simulink model "VSG_AdaptiveJD"  (R2023b)
settings: Solver=ode4  StartTime=0  StopTime=Tsim  FixedStep=Ts  RelTol=1e-3
InitFcn:
  | p0 = fileparts(get_param(bdroot, 'FileName'));
  | if ~isempty(p0), addpath(p0);
  | end;
  | if ~exist('VSG_CASE', 'var'),
  |     VSG_CASE = 'case1';
  | end;
  | if ~exist('VSG_SCHEME', 'var'),
  |     VSG_SCHEME = 5;
  | end;
  | init_vsg_params(VSG_CASE, VSG_SCHEME);
undefined symbols (not defined in the file or in its folder): a_n, b_n, db, delta0, dfref, Dmax, Dmin, dref, DS0, dwref, dzd, dzr, J0, Jmax, Jmin, Kd, kpsi, Kw, lam, lam_floor, muJ, nb, nu, qref, scheme, sigma_n, tau, Ts, txi, w0, wn0, z0, zmax
Description:
  | VSG 转动惯量与阻尼系数协同自适应控制（闭环指标整形, MSCA）
  | 定步长 ode4, Ts = 2e-4 s，与 git/vsg_sim5.py 数值一致。
  | 参数见 init_vsg_params.m；run_vsg_slx.m 复现三工况五方案结果。
settings Model: Creator=Lenovo  LastModifiedBy=Lenovo

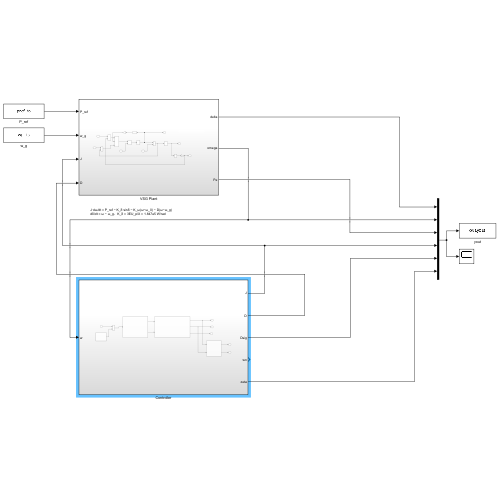
[thumbnail: Simulink's stored preview of the top-level diagram]
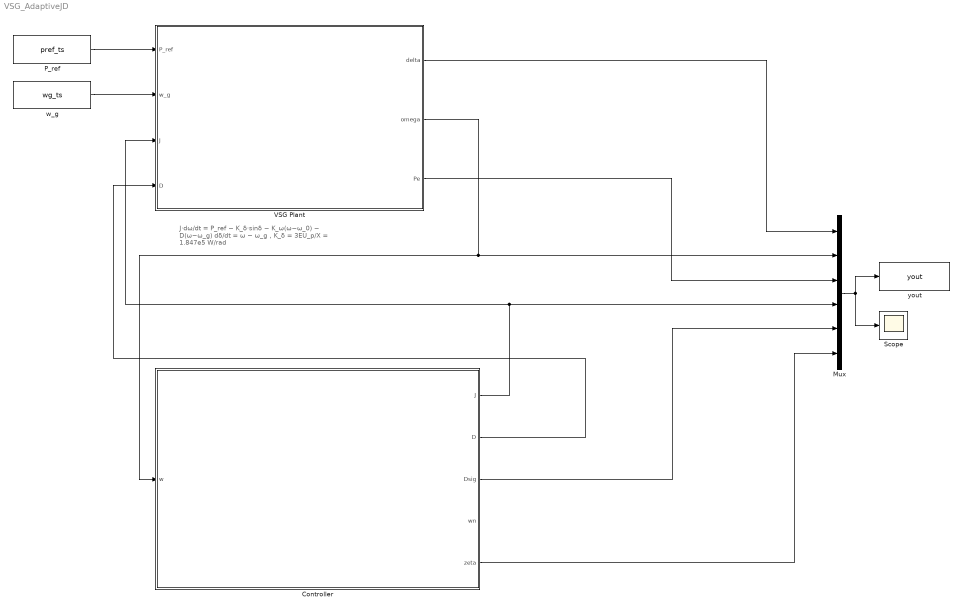
== system VSG_AdaptiveJD ==
  note: J·dω/dt = P_ref − K_δ·sinδ − K_ω(ω−ω_0) − D(ω−ω_g)
      | dδ/dt = ω − ω_g，K_δ = 3EU_p/X = 1.847e5 W/rad
  Controller : Subsystem
  Mux : Mux  Inputs=6
  P_ref : FromWorkspace  VariableName=pref_ts  Interpolate=off  OutputAfterFinalValue=Holding final value
  Scope : Scope
  VSG Plant : Subsystem
  w_g : FromWorkspace  VariableName=wg_ts  Interpolate=off  OutputAfterFinalValue=Holding final value
  yout : ToWorkspace  VariableName=yout  SaveFormat=Timeseries  SampleTime=Ts
  wires:
  P_ref/1 -> VSG Plant/1(P_ref)
  w_g/1 -> VSG Plant/2(w_g)
  VSG Plant/2(omega) -> Controller/1(w), Mux/2
  Controller/1(J) -> VSG Plant/3(J), Mux/4
  Controller/2(D) -> VSG Plant/4(D)
  VSG Plant/1(delta) -> Mux/1
  VSG Plant/3(Pe) -> Mux/3
  Controller/3(Dsig) -> Mux/5
  Controller/5(zeta) -> Mux/6
  Mux/1 -> yout/1, Scope/1

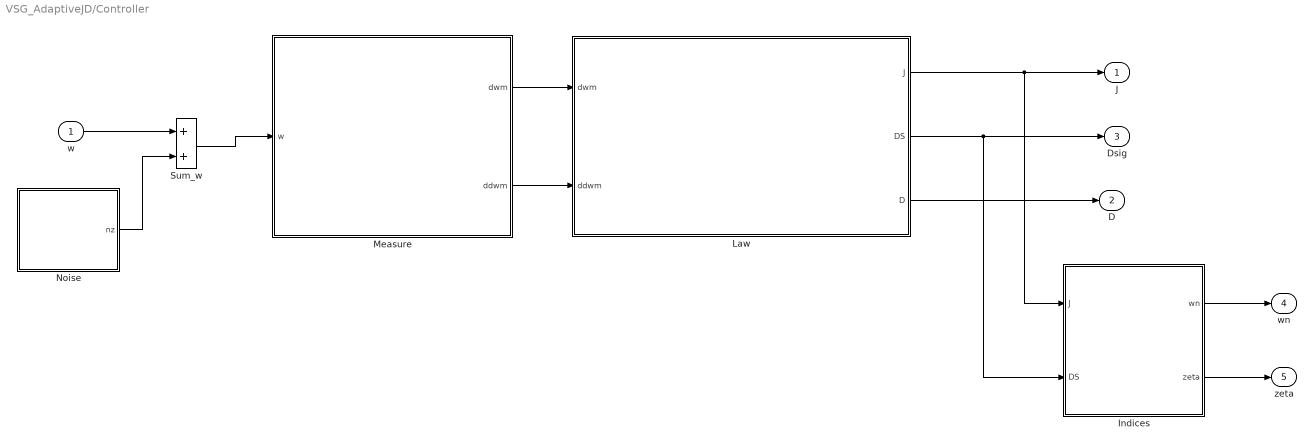
== system VSG_AdaptiveJD/Controller ==
  w : Inport
  Indices : Subsystem
  Law : Subsystem
  Measure : Subsystem
  Noise : Subsystem
  Sum_w : Sum
  J : Outport
  D : Outport  Port=2
  Dsig : Outport  Port=3
  wn : Outport  Port=4
  zeta : Outport  Port=5
  wires:
  w/1 -> Sum_w/1
  Noise/1(nz) -> Sum_w/2
  Sum_w/1 -> Measure/1(w)
  Measure/1(dwm) -> Law/1(dwm)
  Measure/2(ddwm) -> Law/2(ddwm)
  Law/1(J) -> J/1, Indices/1(J)
  Law/2(DS) -> Indices/2(DS), Dsig/1
  Law/3(D) -> D/1
  Indices/1(wn) -> wn/1
  Indices/2(zeta) -> zeta/1

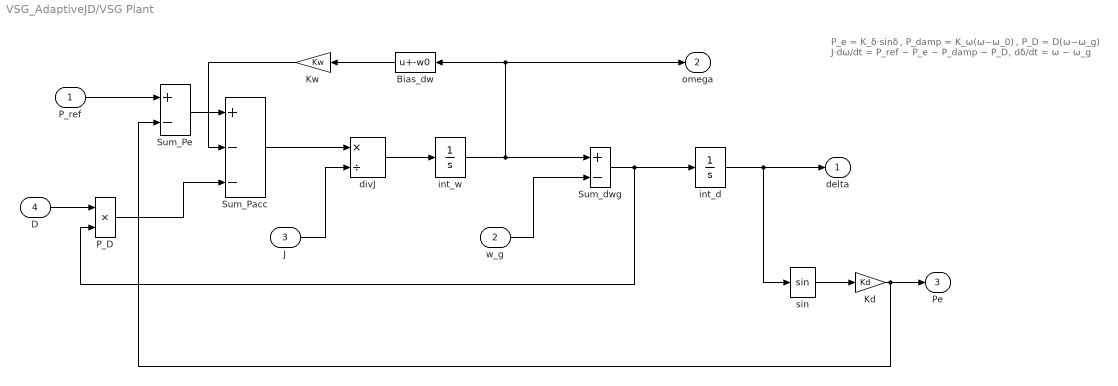
== system VSG_AdaptiveJD/VSG Plant ==
  note: P_e = K_δ·sinδ，P_damp = K_ω(ω−ω_0)，P_D = D(ω−ω_g)
      | J·dω/dt = P_ref − P_e − P_damp − P_D，dδ/dt = ω − ω_g
  P_ref : Inport
  w_g : Inport  Port=2
  J : Inport  Port=3
  D : Inport  Port=4
  Bias_dw : Bias  Bias=-w0  SaturateOnIntegerOverflow=off
  Kd : Gain  Gain=Kd
  Kw : Gain  Gain=Kw
  P_D : Product
  Sum_Pacc : Sum  Inputs=+--
  Sum_Pe : Sum  Inputs=+-
  Sum_dwg : Sum  Inputs=+-
  divJ : Product  Inputs=*/
  int_d : Integrator  InitialCondition=delta0
  int_w : Integrator  InitialCondition=w0
  sin : Trigonometry
  delta : Outport
  omega : Outport  Port=2
  Pe : Outport  Port=3
  wires:
  P_ref/1 -> Sum_Pe/1
  Kd/1 -> Sum_Pe/2, Pe/1
  Sum_Pe/1 -> Sum_Pacc/1
  Kw/1 -> Sum_Pacc/2
  P_D/1 -> Sum_Pacc/3
  Sum_Pacc/1 -> divJ/1
  J/1 -> divJ/2
  divJ/1 -> int_w/1
  int_w/1 -> omega/1, Bias_dw/1, Sum_dwg/1
  Bias_dw/1 -> Kw/1
  w_g/1 -> Sum_dwg/2
  Sum_dwg/1 -> int_d/1, P_D/2
  int_d/1 -> sin/1, delta/1
  sin/1 -> Kd/1
  D/1 -> P_D/1

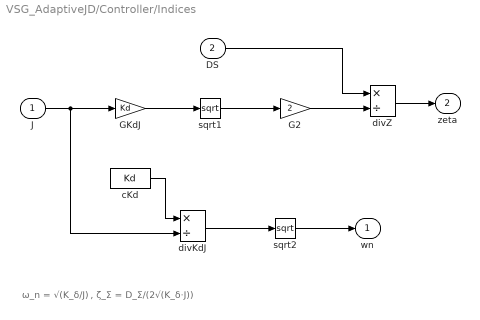
== system VSG_AdaptiveJD/Controller/Indices ==
  note: ω_n = √(K_δ/J)，ζ_Σ = D_Σ/(2√(K_δ·J))
  J : Inport
  DS : Inport  Port=2
  G2 : Gain  Gain=2
  GKdJ : Gain  Gain=Kd
  cKd : Constant  Value=Kd
  divKdJ : Product  Inputs=*/
  divZ : Product  Inputs=*/
  sqrt1 : Sqrt
  sqrt2 : Sqrt
  wn : Outport
  zeta : Outport  Port=2
  wires:
  J/1 -> GKdJ/1, divKdJ/2
  GKdJ/1 -> sqrt1/1
  sqrt1/1 -> G2/1
  cKd/1 -> divKdJ/1
  divKdJ/1 -> sqrt2/1
  sqrt2/1 -> wn/1
  DS/1 -> divZ/1
  G2/1 -> divZ/2
  divZ/1 -> zeta/1

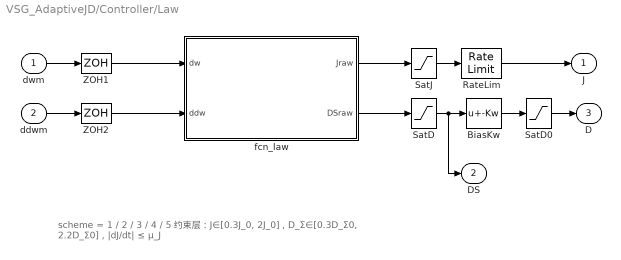
== system VSG_AdaptiveJD/Controller/Law ==
  note: scheme = 1  / 2  / 3  / 4  / 5
      | 约束层：J∈[0.3J_0, 2J_0]，D_Σ∈[0.3D_Σ0, 2.2D_Σ0]，|dJ/dt| ≤ μ_J
  dwm : Inport
  ddwm : Inport  Port=2
  BiasKw : Bias  Bias=-Kw  SaturateOnIntegerOverflow=off
  RateLim : RateLimiter  RisingSlewLimit=muJ  FallingSlewLimit=-muJ  SampleTimeMode=inherited  InitialCondition=J0
  SatD : Saturate  UpperLimit=Dmax  LowerLimit=Dmin
  SatD0 : Saturate  UpperLimit=inf  LowerLimit=0
  SatJ : Saturate  UpperLimit=Jmax  LowerLimit=Jmin
  ZOH1 : ZeroOrderHold  SampleTime=Ts
  ZOH2 : ZeroOrderHold  SampleTime=Ts
  fcn_law : MATLAB Function  TreatAsAtomicUnit=on
  J : Outport
  DS : Outport  Port=2
  D : Outport  Port=3
  wires:
  dwm/1 -> ZOH1/1
  ddwm/1 -> ZOH2/1
  ZOH1/1 -> fcn_law/1(dw)
  ZOH2/1 -> fcn_law/2(ddw)
  fcn_law/1(Jraw) -> SatJ/1
  SatJ/1 -> RateLim/1
  RateLim/1 -> J/1
  fcn_law/2(DSraw) -> SatD/1
  SatD/1 -> BiasKw/1, DS/1
  BiasKw/1 -> SatD0/1
  SatD0/1 -> D/1

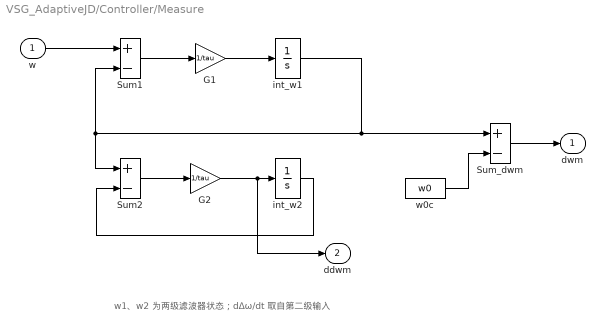
== system VSG_AdaptiveJD/Controller/Measure ==
  note: w1、w2 为两级滤波器状态；dΔω/dt 取自第二级输入
  w : Inport
  G1 : Gain  Gain=1/tau
  G2 : Gain  Gain=1/tau
  Sum1 : Sum  Inputs=+-
  Sum2 : Sum  Inputs=+-
  Sum_dwm : Sum  Inputs=+-
  int_w1 : Integrator  InitialCondition=w0
  int_w2 : Integrator  InitialCondition=w0
  w0c : Constant  Value=w0
  dwm : Outport
  ddwm : Outport  Port=2
  wires:
  w/1 -> Sum1/1
  int_w1/1 -> Sum2/1, Sum1/2, Sum_dwm/1
  Sum1/1 -> G1/1
  G1/1 -> int_w1/1
  int_w2/1 -> Sum2/2
  Sum2/1 -> G2/1
  G2/1 -> ddwm/1, int_w2/1
  w0c/1 -> Sum_dwm/2
  Sum_dwm/1 -> dwm/1

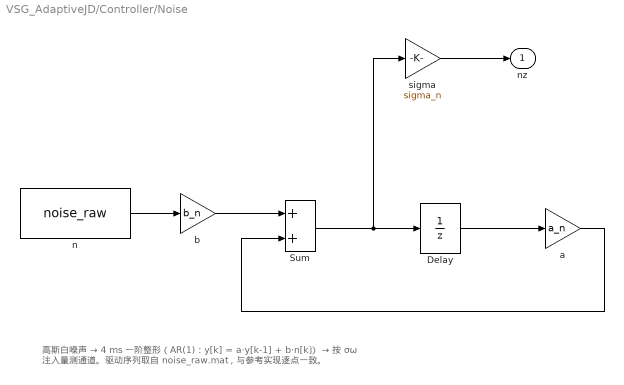
== system VSG_AdaptiveJD/Controller/Noise ==
  note: 高斯白噪声 → 4 ms 一阶整形（AR(1)：y[k] = a·y[k-1] + b·n[k]）
      | → 按 σω 注入量测通道。驱动序列取自 noise_raw.mat，与参考实现逐点一致。
  Delay : UnitDelay  SampleTime=Ts  HasFrameUpgradeWarning=on
  Sum : Sum
  a : Gain  Gain=a_n
  b : Gain  Gain=b_n
  n : FromWorkspace  VariableName=noise_raw  SampleTime=Ts  Interpolate=off  OutputAfterFinalValue=Holding final value
  sigma : Gain  Gain=sigma_n
  nz : Outport
  wires:
  n/1 -> b/1
  b/1 -> Sum/1
  Sum/1 -> sigma/1, Delay/1
  Delay/1 -> a/1
  a/1 -> Sum/2
  sigma/1 -> nz/1

== matlab function VSG_AdaptiveJD/Controller/Law/fcn_law ==
  data: dw input; Jraw output; ddw input; DSraw output; qref parameter; J0 parameter; DS0 parameter; dfref parameter; dwref parameter; dref parameter; txi parameter; Ts parameter; kpsi parameter; db parameter; wn0 parameter; nu parameter; nb parameter; z0 parameter; dzr parameter; dzd parameter; lam parameter; zmax parameter; Kd parameter; scheme parameter; lam_floor parameter
function [Jraw, DSraw] = fcn_law(dw, ddw, qref, J0, DS0, dfref, dwref, dref, txi, Ts, kpsi, db, wn0, nu, nb, z0, dzr, dzd, lam, zmax, Kd, scheme, lam_floor)



% scheme = 1 Fixed / 2 Exponential / 3 antitangent / 4 segmentation / 5 MSCA

persistent xf

if isempty(xf)

    xf = 0;

end

xi = dw*ddw/max(qref, 1e-9);

Jraw = J0;

DSraw = DS0;

switch scheme

    case 1                      % S1 

        Jraw  = J0;

        DSraw = DS0;

    case 2                      % S2 ：D_Sigma = sqrt(C*J)

        r = abs(ddw)/(2*pi)/max(dfref, 1e-9);

        Jraw  = J0*(1 + r^2);

        DSraw = DS0*sqrt(Jraw/J0);

    case 3                      % S3 

        xd = 0.05;

        if xi >= xd

            Jraw = J0 + (2*J0/pi)*atan(1.1*(xi - xd));

        elseif xi <= -xd

            Jraw = J0 + (2*J0/pi)*atan(1.1*(xi + xd));

        else

            Jraw = J0;

        end

        if abs(dw) > 0.03*dwref

            DSraw = DS0 + 0.45*DS0/dwref*abs(dw) + 0.10*DS0/dref*abs(ddw);

        else

            DSraw = DS0;

        end

    case 4                      % S4 

        q  = abs(ddw)*abs(dw)/max(qref, 1e-9);

        if dw*ddw > 0

            sg = 1;

        else

            sg = -1;

        end

        Jraw  = J0 + sg*J0*q;

        DSraw = DS0 - sg*0.55*11*J0*q;

    otherwise                   % S5 MSCA

        if txi > 0

            xf = xf + (xi - xf)*Ts/txi;   

            xi = xf;

        end

        s  = (2/pi)*atan(kpsi*(xi - db*tanh(xi/db)));  

        sp = max(s, 0);

        sm = min(s, 0);

        wn = wn0*(1 - nu*sp - nb*sm);                 

        zs = z0 + dzd*sp - dzr*sm;                    

        if lam_floor > 0

            zf = lam/wn;

        else

            zf = z0;

        end

        z = min(max(max(zs, zf), z0), zmax);

        Jraw  = Kd/wn^2;                              

        DSraw = 2*z*sqrt(Kd*Jraw);                    

end

end
